simulink model "L2_scheme"  (R2023b)
settings: Solver=VariableStepAuto  StartTime=0.0  StopTime=10.0  RelTol=1e-3
settings Model: Creator=Admin  LastModifiedBy=Admin

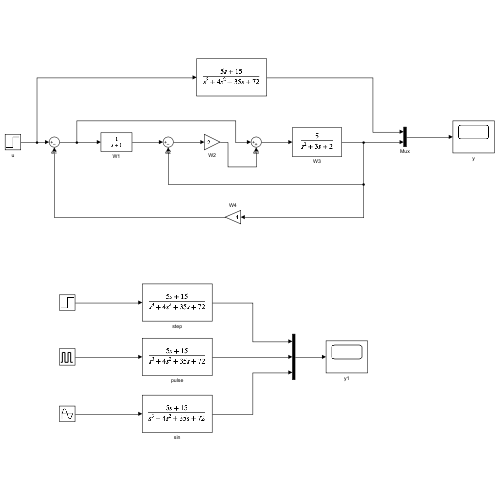
[thumbnail: Simulink's stored preview of the top-level diagram]
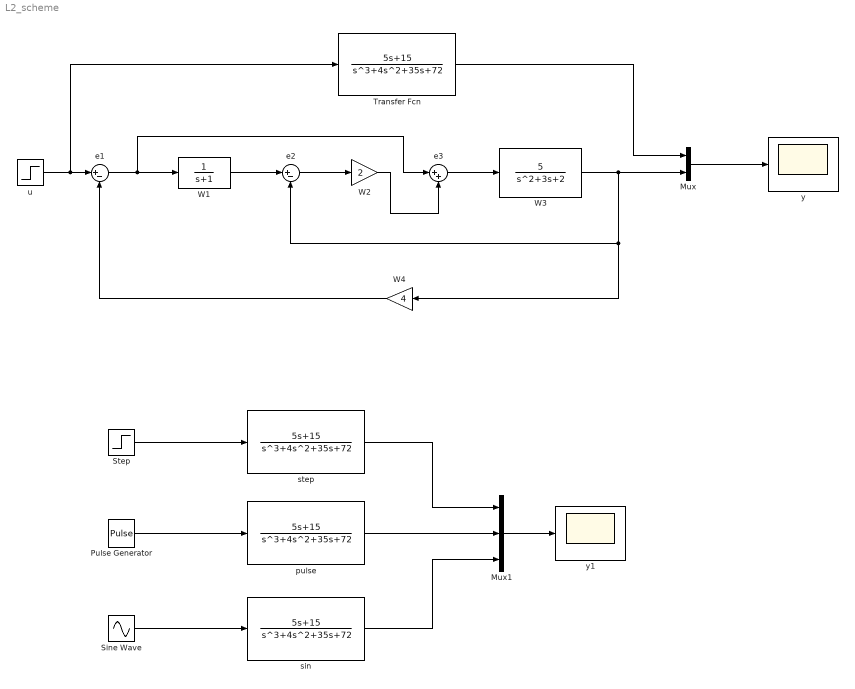
== system L2_scheme ==
  Mux : Mux  Inputs=2
  Mux1 : Mux  Inputs=3
  Pulse Generator : DiscretePulseGenerator  PulseType=Time based  Period=10  PulseWidth=5
  Sine Wave : Sin  SampleTime=0
  Step : Step  SampleTime=0
  Transfer Fcn : TransferFcn  Numerator=[5 15]  Denominator=[1 4 35 72]
  W1 : TransferFcn  Denominator=[1 1]  ContinuousStateAttributes="\"\""
  W2 : Gain  Gain=2
  W3 : TransferFcn  Numerator=[5]  Denominator=[1 3 2]
  W4 : Gain  Gain=4
  e1 : Sum  Inputs=|+-
  e2 : Sum  Inputs=|+-
  e3 : Sum  Inputs=|++
  pulse : TransferFcn  Numerator=[5 15]  Denominator=[1 4 35 72]
  sin : TransferFcn  Numerator=[5 15]  Denominator=[1 4 35 72]
  step : TransferFcn  Numerator=[5 15]  Denominator=[1 4 35 72]
  u : Step  SampleTime=0
  y : Scope
  y1 : Scope
  wires:
  u/1 -> Transfer Fcn/1, e1/1
  e1/1 -> e3/1, W1/1
  W1/1 -> e2/1
  e2/1 -> W2/1
  W2/1 -> e3/2
  e3/1 -> W3/1
  W3/1 -> Mux/2, e2/2, W4/1
  W4/1 -> e1/2
  Mux/1 -> y/1
  Transfer Fcn/1 -> Mux/1
  step/1 -> Mux1/1
  pulse/1 -> Mux1/2
  sin/1 -> Mux1/3
  Sine Wave/1 -> sin/1
  Pulse Generator/1 -> pulse/1
  Step/1 -> step/1
  Mux1/1 -> y1/1
